simulink model "Grid_ModelSim2AEMO3Phasefaultincluded"  (R2025a)
settings: Solver=daessc  StartTime=0.0  StopTime=50  RelTol=1e-3
InitFcn:
  | Grid_ModelSimV1
values from neighbouring files (symbols this model uses):
  D2 = 3    [Grid_ModelSimV1.m]
  E1_0 = 1.0    (= 1)    [Grid_ModelSimV1.m]
  E2_0 = 1.0    (= 1)    [Grid_ModelSimV1.m]
  H1 = 3    [Grid_ModelSimV1.m]
  H2 = 5    [Grid_ModelSimV1.m]
  Pm1 = 0.8    [Grid_ModelSimV1.m]
  ws = 2*pi*f    (= 314.159265359)    [Grid_ModelSimV1.m]
libraries: ee_lib x7, nesl_utility x7, fl_lib x2, eePowerMeasurement x1
settings Model: Creator=DavidBore  LastModifiedBy=DavidBore

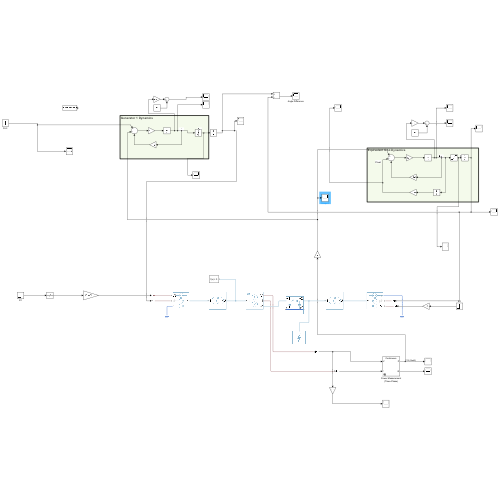
[thumbnail: Simulink's stored preview of the top-level diagram]
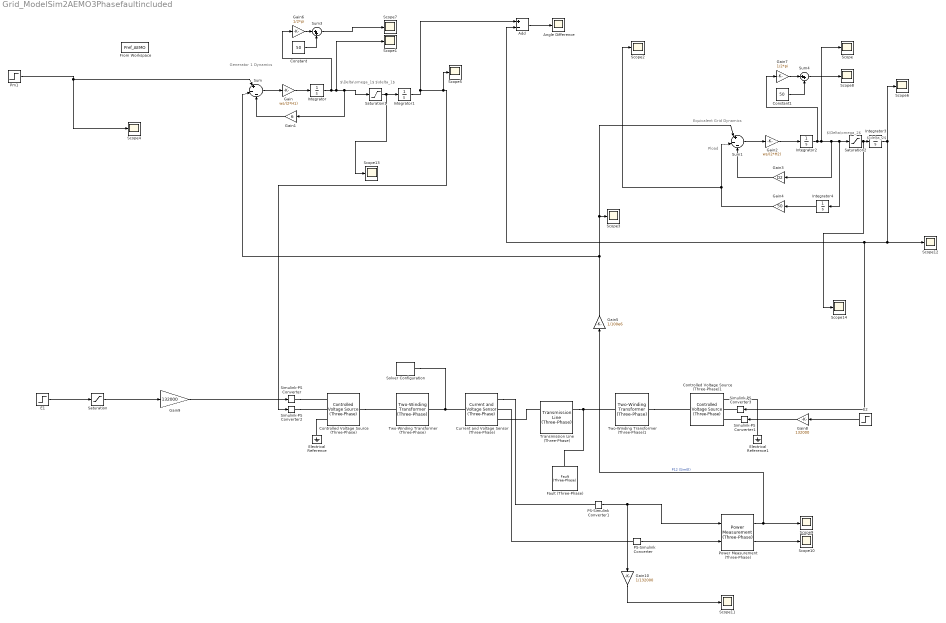
== system Grid_ModelSim2AEMO3Phasefaultincluded ==
  note: Pload
  note: Equivalent Grid Dynamics
  note: $\delta_1$
  note: $\Delta\omega_1$
  note: Generator 1 Dynamics
  note: $\Delta\omega_2$
  note: $\delta_2$
  Add : Sum  Inputs=+-
  Angle Difference : Scope
      settings: ActiveDisplayYMinimum=-0.0716976723273877  ActiveDisplayYMaximum=0.64527905094648941  DataLoggingVariableName=ScopeData11
  Constant : Constant  Value=50
  Constant1 : Constant  Value=50
  Controlled Voltage Source (Three-Phase) : ee_lib/Sources/Controlled Voltage Source (Three-Phase)  input_option=ee.enum.inputType.singleFreqAC  FRated=50 Hz
      settings: InternalSimscapePortConfiguration="{\"Bottom\":[],\"Left\":[{\"id\":\"Vt\",\"label\":\"Vt\",\"type\":\"input\"},{\"id\":\"ph\",\"label\":\"ph\",\"type\":\"input\"},{\"id\":\"n\",\"label\":\"n\",\"type\":\"foundation.electrical.electrical\"}],\"Right\":[{\"id\":\"N\",\"label\":\"~\",\"type\":\"foundation.electrical.three_phase\"}],\"Top\":[]}"
  Controlled Voltage Source (Three-Phase)1 : ee_lib/Sources/Controlled Voltage Source (Three-Phase)  input_option=ee.enum.inputType.singleFreqAC  FRated=50 Hz
      settings: InternalSimscapePortConfiguration="{\"Bottom\":[],\"Left\":[{\"id\":\"Vt\",\"label\":\"Vt\",\"type\":\"input\"},{\"id\":\"ph\",\"label\":\"ph\",\"type\":\"input\"},{\"id\":\"n\",\"label\":\"n\",\"type\":\"foundation.electrical.electrical\"}],\"Right\":[{\"id\":\"N\",\"label\":\"~\",\"type\":\"foundation.electrical.three_phase\"}],\"Top\":[]}"
  Current and Voltage Sensor (Three-Phase) : ee_lib/Sensors & Transducers/Current and Voltage Sensor (Three-Phase)  vMeasurementType=ee.enum.vmeasurement.ll  outputUnit=ee.enum.unit.si  SRated=100e6 A*V  VRated=24e3 V  I_specify=off  I_priority=None  I=[0, 0, 0] A  I_nominal_specify=off  I_nominal_value=1  I_nominal_unit=A  V_specify=off  V_priority=None  V=[0, 0, 0] V  V_nominal_specify=off  V_nominal_value=1  V_nominal_unit=V
      settings: InternalSimscapePortConfiguration="{\"Bottom\":[],\"Left\":[{\"id\":\"N1\",\"label\":\"~1\",\"type\":\"foundation.electrical.three_phase\"}],\"Right\":[{\"id\":\"V_output\",\"label\":\"V\",\"type\":\"output\"},{\"id\":\"I_output\",\"label\":\"I\",\"type\":\"output\"},{\"id\":\"N2\",\"label\":\"~2\",\"type\":\"foundation.electrical.three_phase\"}],\"Top\":[]}"
  E1 : Step  Before=E1_0  After=E1_0  SampleTime=0
  E2 : Step  Before=E2_0  After=E2_0  SampleTime=0
  Electrical Reference : fl_lib/Electrical/Electrical Elements/Electrical Reference
  Electrical Reference1 : fl_lib/Electrical/Electrical Elements/Electrical Reference
  Fault (Three-Phase) : ee_lib/Utilities/Fault (Three-Phase)  fault_type_option=11  R_pn_fault=1e-3 Ohm  R_ng_fault=1e-3 Ohm  exposemeasurement=ee.enum.exposemeasurement.hidden  enable_external_fault=ee.enum.external_fault.hidden  fault_threshold=0.5  fault_condition=1  fault_resettable=0  enable_temporal_fault=1  fault_start_time=5 s  fault_duration=0.43 s  G_parasitic=1e-6 1/Ohm
      settings: InternalSimscapePortConfiguration="{\"Bottom\":[],\"Left\":[{\"id\":\"N\",\"label\":\"~\",\"type\":\"foundation.electrical.three_phase\"}],\"Right\":[],\"Top\":[]}"
  From Workspace : FromWorkspace  VariableName=Pref_AEMO  Interpolate=off  OutputAfterFinalValue=Holding final value
  Gain : Gain  Gain=ws/(2*H1)
  Gain1 : Gain  Gain=6
  Gain10 : Gain  Gain=1/132000
  Gain2 : Gain  Gain=ws/(2*H2)
  Gain3 : Gain  Gain=D2
  Gain4 : Gain  Gain=50
  Gain5 : Gain  Gain=1/100e6
  Gain6 : Gain  Gain=1/2*pi
  Gain7 : Gain  Gain=1/2*pi
  Gain8 : Gain  Gain=132000
  Gain9 : Gain  Gain=132000
  Integrator{,1..4} (5 alike) : Integrator
  PS-Simulink Converter : nesl_utility/PS-Simulink Converter  PhysicalDomain=network_engine_domain  SubClassName=ps_output  LeftPortType=input  RightPortType=output  PseudoPeriodic=off  Frequencies=[]  VectorFormat=inherit  Unit=inherit  AffineConversion=off
  PS-Simulink Converter1 : nesl_utility/PS-Simulink Converter  PhysicalDomain=network_engine_domain  SubClassName=ps_output  LeftPortType=input  RightPortType=output  PseudoPeriodic=off  Frequencies=[]  VectorFormat=inherit  Unit=inherit  AffineConversion=off
  Pm1 : Step  Time=5  Before=Pm1  After=Pm1  SampleTime=0
  Power Measurement (Three-Phase) : eePowerMeasurement/Power Measurement (Three-Phase)  LabelModeActiveChoice=Continuous  F=50  K=1  Seq=Positive  Ts=0
  Saturation : Saturate  UpperLimit=1.1  LowerLimit=0.9
  Saturation1 : Saturate  UpperLimit=0.02  LowerLimit=-0.02
  Saturation2 : Saturate  UpperLimit=0.2  LowerLimit=-0.2
  Scope{,1..14} (15 alike) : Scope
      Scope10 settings: ActiveDisplayYMinimum=-3.79328240985179E+8  ActiveDisplayYMaximum=4.1955305631289077E+8  DataLoggingVariableName=ScopeData10
      Scope11 settings: ActiveDisplayYMinimum=-288.17448446172642  ActiveDisplayYMaximum=124.86295167484585  DataLoggingVariableName=ScopeData12
      Scope12 settings: ActiveDisplayYMinimum=-0.32102755309126052  ActiveDisplayYMaximum=0.30164178337724734  DataLoggingVariableName=ScopeData13
      Scope13 settings: ActiveDisplayYMinimum=-0.21710171878509654  ActiveDisplayYMaximum=0.51220748739382271  DataLoggingVariableName=ScopeData14
      Scope14 settings: ActiveDisplayYMinimum=-0.25  ActiveDisplayYMaximum=0.25  DataLoggingVariableName=ScopeData15
      Scope2 settings: ActiveDisplayYMinimum=-1.1623447136135812  ActiveDisplayYMaximum=1.3781315704633705  DataLoggingVariableName=ScopeData2
      Scope3 settings: ActiveDisplayYMinimum=-1.7945921446279036  ActiveDisplayYMaximum=1.4876121145303298  DataLoggingVariableName=ScopeData3
      Scope4 settings: ActiveDisplayYMinimum=0.32151036058031318  ActiveDisplayYMaximum=1.2098623971073263  DataLoggingVariableName=ScopeData4
      Scope5 settings: ActiveDisplayYMinimum=-0.15499931008114687  ActiveDisplayYMaximum=1.3546102723832139  DataLoggingVariableName=ScopeData5
      Scope6 settings: ActiveDisplayYMinimum=-0.32102755309126052  ActiveDisplayYMaximum=0.30164178337724734  DataLoggingVariableName=ScopeData6
      Scope7 settings: ActiveDisplayYMinimum=48.472996051879186  ActiveDisplayYMaximum=52.414974467711623  DataLoggingVariableName=ScopeData7
      Scope8 settings: ActiveDisplayYMinimum=49.92788610274394  ActiveDisplayYMaximum=50.170097472488152  DataLoggingVariableName=ScopeData8
      Scope9 settings: ActiveDisplayYMinimum=-1.1545760941367698E+8  ActiveDisplayYMaximum=4.164743531344825E+8  DataLoggingVariableName=ScopeData9
  Simulink-PS Converter{,1..3} (4 alike) : nesl_utility/Simulink-PS Converter  PhysicalDomain=network_engine_domain  SubClassName=ps_input  LeftPortType=input  RightPortType=output  PseudoPeriodic=off  Frequencies=[]  NoiseDistribution=none  NoiseParameters=[]  Unit=1  AffineConversion=off  FilteringAndDerivatives=provide  SimscapeFilterOrder=1  InputFilterTimeConstant=0.001  UdotUserProvided=0
  Solver Configuration : nesl_utility/Solver Configuration  PhysicalDomain=network_engine_domain  SubClassName=solver  LeftPortType=input  RightPortType=generic  Tones=[]  Harmonics=[]  SimulateNoise=off  Profile=off  UseLocalSampling=off  EnableSwitchedLinearOptims=on  FrequencyDomain=off  UseCCode=off  RelTol=0.001  AbsTol=0.001  MinStep=1e-09  ToWorkspace=off  RevertToSquareIcSolve=off  NumHomotopyIterations=100  PhasorMode=off  PhasorModeNumHarmonics=1  ConsistencySolver=NEWTON_XTOL_AFTER_FTOL  IndexReductionMethod=DerivativeReplacement  DoDC=off  ResidualTolerance=1e-09  ConsistencyTolSource=GLOBAL  ConsistencyAbsTol=0.001  ConsistencyRelTol=0.001  ConsistencyTolFactor=0.001  UseLocalSolver=off  LocalSolverChoice=NE_BACKWARD_EULER_ADVANCER  ResolveIndetEquations=on  FunctionEvalNumThread=1  LocalSolverSampleTime=0.001  DoFixedCost=off  MaxNonlinIter=3  MaxModeIter=2  ComputeImpulses=off  ImpulseIterations=2  LinearAlgebra=auto  LinearAlgebraNumThread=0  EquationFormulation=NE_TIME_EF  DelaysMemoryBudget=1024  AutomaticFiltering=on  FilteringTimeConstant=0.001  PartitionStorageMethod=AS_NEEDED  PartitionMemoryBudget=1024  PartitionMethod=ROBUST  MultibodyUseLocalSolver=off  MultibodyLocalSolverChoice=ODE1  MultibodyLocalSolverSampleTime=0.001
  Sum : Sum  Inputs=|+|-|-
  Sum1 : Sum  Inputs=|+|-|-
  Sum3 : Sum  Inputs=|++
  Sum4 : Sum  Inputs=|++
  Transmission Line (Three-Phase) : ee_lib/Passive/Lines/Transmission Line (Three-Phase)  length=1 km  freq=50 Hz  R=0.01 Ohm/km  L=55.46 mH/km  M=0 mH/km  Cl=0.3 uF/km  Cg=0.1 uF/km  Rm=0 Ohm/km  ModelTwoSections=ee.enum.enable.no  N=1  InterfacePosition=0.5 km  N1sec=1  N2sec=1  Access_ground=ee.enum.enable.no  R_parasitic=1e-6 Ohm  G_parasitic=1e-6 1/Ohm
      settings: InternalSimscapePortConfiguration="{\"Bottom\":[],\"Left\":[{\"id\":\"N1\",\"label\":\"~1\",\"type\":\"foundation.electrical.three_phase\"},{\"id\":\"g1\",\"label\":\"g1\",\"type\":\"foundation.electrical.electrical\"}],\"Right\":[{\"id\":\"N2\",\"label\":\"~2\",\"type\":\"foundation.electrical.three_phase\"},{\"id\":\"g2\",\"label\":\"g2\",\"type\":\"foundation.electrical.electrical\"}],\"Top\":[]}"
  Two-Winding Transformer (Three-Phase) : ee_lib/Passive/Transformers/Two-Winding Transformer (Three-Phase)  SRated=100e6 A*V  FRated=50 Hz  Winding1Connection=ee.enum.windingconnection.Yg  VRated1=132000 V  Winding2Connection=ee.enum.windingconnection.Yg  VRated2=132000 V  CoreType=ee.enum.coretype.threelimb  pu_Rw1=0.001  pu_Rw2=0.001  leakage_reactance_option=ee.enum.transformer_leakage.include  pu_Xl1=0.075  pu_Xl2=0.075  magnetizing_resistance_option=ee.enum.transformer_magnetizingResistance.exclude  pu_Rm=500  magnetizing_reactance_option=ee.enum.transformer_magnetizingReactance.exclude  saturation_option=ee.enum.transformer_saturation.exclude  pu_Xm=500  current_data=[0, .002, 1, 2]  magnetic_flux_data=[0, 1.2, 1.5, 1.51]  pu_X0=0.5  i1_specify=off  i1_priority=None  i1=[0, 0, 0] A  i1_nominal_specify=off  i1_nominal_value=1  i1_nominal_unit=A  i2_specify=off  i2_priority=None  i2=[0, 0, 0] A  i2_nominal_specify=off  i2_nominal_value=1  i2_nominal_unit=A  phi_specify=off  phi_priority=None  phi=[0, 0, 0]  phi_nominal_specify=off  phi_nominal_value=1  phi_nominal_unit=1  power_dissipated_specify=off  power_dissipated_priority=None  power_dissipated=0 W  power_dissipated_nominal_specify=off  power_dissipated_nominal_value=1  power_dissipated_nominal_unit=W
      settings: InternalSimscapePortConfiguration="{\"Bottom\":[],\"Left\":[{\"id\":\"N1\",\"label\":\"~1\",\"type\":\"foundation.electrical.three_phase\"}],\"Right\":[{\"id\":\"N2\",\"label\":\"~2\",\"type\":\"foundation.electrical.three_phase\"}],\"Top\":[]}"
  Two-Winding Transformer (Three-Phase)1 : ee_lib/Passive/Transformers/Two-Winding Transformer (Three-Phase)  SRated=100e6 A*V  FRated=50 Hz  Winding1Connection=ee.enum.windingconnection.Y  VRated1=132000 V  Winding2Connection=ee.enum.windingconnection.Y  VRated2=132000 V  CoreType=ee.enum.coretype.threelimb  pu_Rw1=0.001  pu_Rw2=0.001  leakage_reactance_option=ee.enum.transformer_leakage.include  pu_Xl1=0.075  pu_Xl2=0.075  magnetizing_resistance_option=ee.enum.transformer_magnetizingResistance.exclude  pu_Rm=500  magnetizing_reactance_option=ee.enum.transformer_magnetizingReactance.exclude  saturation_option=ee.enum.transformer_saturation.exclude  pu_Xm=500  current_data=[0, .002, 1, 2]  magnetic_flux_data=[0, 1.2, 1.5, 1.51]  pu_X0=0.5  i1_specify=off  i1_priority=None  i1=[0, 0, 0] A  i1_nominal_specify=off  i1_nominal_value=1  i1_nominal_unit=A  i2_specify=off  i2_priority=None  i2=[0, 0, 0] A  i2_nominal_specify=off  i2_nominal_value=1  i2_nominal_unit=A  phi_specify=off  phi_priority=None  phi=[0, 0, 0]  phi_nominal_specify=off  phi_nominal_value=1  phi_nominal_unit=1  power_dissipated_specify=off  power_dissipated_priority=None  power_dissipated=0 W  power_dissipated_nominal_specify=off  power_dissipated_nominal_value=1  power_dissipated_nominal_unit=W
      settings: InternalSimscapePortConfiguration="{\"Bottom\":[],\"Left\":[{\"id\":\"N1\",\"label\":\"~1\",\"type\":\"foundation.electrical.three_phase\"}],\"Right\":[{\"id\":\"N2\",\"label\":\"~2\",\"type\":\"foundation.electrical.three_phase\"}],\"Top\":[]}"
  wires:
  Pm1/1 -> Sum/1, Scope4/1
  Sum/1 -> Gain/1
  Gain/1 -> Integrator/1
  Integrator/1 -> Gain6/1, Scope1/1, Gain1/1, Saturation1/1
  Gain1/1 -> Sum/3
  Sum1/1 -> Gain2/1
  Integrator2/1 -> Gain7/1, Scope/1, Saturation2/1, Integrator4/1, Gain3/1
  Gain2/1 -> Integrator2/1
  Gain3/1 -> Sum1/3
  Integrator4/1 -> Gain4/1
  Gain4/1 -> Scope2/1, Sum1/2
  E1/1 -> Saturation/1
  Gain6/1 -> Sum3/1
  Gain7/1 -> Sum4/1
  Constant/1 -> Sum3/2
  Constant1/1 -> Sum4/2
  Sum3/1 -> Scope7/1
  Sum4/1 -> Scope8/1
  PS-Simulink Converter1/1 -> Power Measurement (Three-Phase)/1, Gain10/1
  PS-Simulink Converter/1 -> Power Measurement (Three-Phase)/2
  Power Measurement (Three-Phase)/2 -> Scope10/1
  E2/1 -> Gain8/1
  Power Measurement (Three-Phase)/1 -> Scope9/1, Gain5/1  "P12 (SimEl)"
  Gain8/1 -> Simulink-PS Converter1/1
  Gain5/1 -> Sum1/1, Scope3/1, Sum/2
  Add/1 -> Angle Difference/1
  Gain10/1 -> Scope11/1
  Gain9/1 -> Simulink-PS Converter/1
  Saturation/1 -> Gain9/1
  Integrator1/1 -> Add/1, Scope5/1, Simulink-PS Converter2/1
  Integrator3/1 -> Scope12/1, Add/2, Simulink-PS Converter3/1, Scope6/1
  Saturation1/1 -> Scope13/1, Integrator1/1
  Saturation2/1 -> Scope14/1, Integrator3/1
  connections:
  Controlled Voltage Source (Three-Phase)/RConn1 -- Two-Winding Transformer (Three-Phase)/LConn1
  Transmission Line (Three-Phase)/RConn1 -- Two-Winding Transformer (Three-Phase)1/LConn1 -- Fault (Three-Phase)/LConn1
  Electrical Reference/LConn1 -- Controlled Voltage Source (Three-Phase)/LConn3
  Electrical Reference1/LConn1 -- Controlled Voltage Source (Three-Phase)1/LConn3
  Two-Winding Transformer (Three-Phase)1/RConn1 -- Controlled Voltage Source (Three-Phase)1/RConn1
  Simulink-PS Converter3/RConn1 -- Controlled Voltage Source (Three-Phase)1/LConn2
  Current and Voltage Sensor (Three-Phase)/RConn1 -- PS-Simulink Converter1/LConn1
  PS-Simulink Converter/LConn1 -- Current and Voltage Sensor (Three-Phase)/RConn2
  Simulink-PS Converter/RConn1 -- Controlled Voltage Source (Three-Phase)/LConn1
  Simulink-PS Converter2/RConn1 -- Controlled Voltage Source (Three-Phase)/LConn2
  Simulink-PS Converter1/RConn1 -- Controlled Voltage Source (Three-Phase)1/LConn1
  Current and Voltage Sensor (Three-Phase)/LConn1 -- Solver Configuration/RConn1 -- Two-Winding Transformer (Three-Phase)/RConn1
  Transmission Line (Three-Phase)/LConn1 -- Current and Voltage Sensor (Three-Phase)/RConn3
